simulink model "cbs_sim"  (R2023b)
settings: Solver=FixedStepDiscrete  StartTime=0.0  StopTime=(1e6-1)*Tb  FixedStep=Tb  RelTol=1e-3
undefined symbols (not defined in the file): graine, p1, pe, Tb
settings Model: Creator=e2507457  LastModifiedBy=e2507457

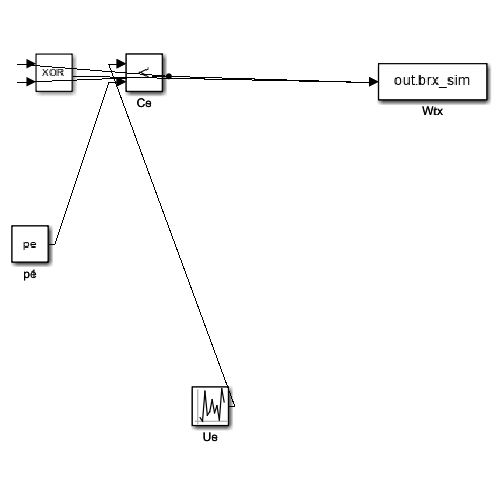
[thumbnail: Simulink's stored preview of the top-level diagram]
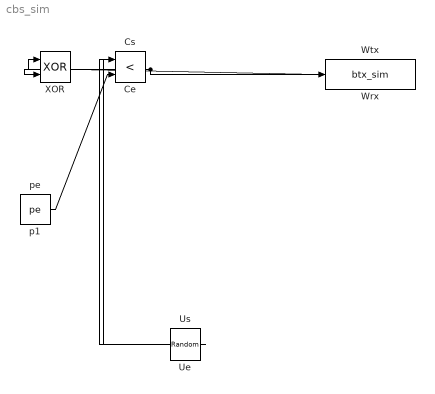
== system cbs_sim ==
  Ce : RelationalOperator  Operator=<  OutDataTypeStr=boolean  RndMeth=Simplest  InputSameDT=off
  Cs : RelationalOperator  Operator=<  OutDataTypeStr=boolean  RndMeth=Simplest  InputSameDT=off
  Ue : UniformRandomNumber  Minimum=0  Seed=graine+1  SampleTime=Tb
  Us : UniformRandomNumber  Minimum=0  Seed=graine  SampleTime=Tb
  Wrx : ToWorkspace  VariableName=brx_sim  SampleTime=-1
  Wtx : ToWorkspace  VariableName=btx_sim  SampleTime=-1
  XOR : Logic  Operator=XOR  AllPortsSameDT=off  OutDataTypeStr=boolean
  p1 : Constant  Value=p1  SampleTime=Tb
  pe : Constant  Value=pe  SampleTime=Tb
  wires:
  Us/1 -> Cs/1
  p1/1 -> Cs/2
  Ue/1 -> Ce/1
  pe/1 -> Ce/2
  Cs/1 -> XOR/1, Wtx/1
  Ce/1 -> XOR/2
  XOR/1 -> Wrx/1
